simulink model "Lab2_Task_1"  (R2026a)
settings: Solver=FixedStepAuto  StopTime=inf
model workspace (MAT data in the model file):
  SL_ROS_VariableLengthArrays_MaxSizes.CommonInfo.ArrayTruncateAction = 'EmitWarning'
  SL_ROS_VariableLengthArrays_MaxSizes.MsgTypeMap = containers.Map
  SL_ROS_VariableLengthArrays_MaxSizes.MsgTypeMap.serialization.keys = {'sensor_msgs/LaserScan'}
  SL_ROS_VariableLengthArrays_MaxSizes.MsgTypeMap.serialization.values{1}(1).PropertyName = 'intensities'
  SL_ROS_VariableLengthArrays_MaxSizes.MsgTypeMap.serialization.values{1}(1).DataType = 'single'
  SL_ROS_VariableLengthArrays_MaxSizes.MsgTypeMap.serialization.values{1}(1).MaxLength = 360
  SL_ROS_VariableLengthArrays_MaxSizes.MsgTypeMap.serialization.values{1}(2).PropertyName = 'ranges'
  SL_ROS_VariableLengthArrays_MaxSizes.MsgTypeMap.serialization.values{1}(2).DataType = 'single'
  SL_ROS_VariableLengthArrays_MaxSizes.MsgTypeMap.serialization.values{1}(2).MaxLength = 360
  SL_ROS_VariableLengthArrays_MaxSizes.MsgTypeMap.serialization.uniformity = 0
  SL_ROS_VariableLengthArrays_MaxSizes.MsgTypeMap.serialization.keyType = 'char'
  SL_ROS_VariableLengthArrays_MaxSizes.MsgTypeMap.serialization.valueType = 'any'
undefined symbols (not defined in the file): header, twist
libraries: ros2lib x4
settings Model: Creator=scott  LastModifiedBy=juulg
settings OptimizationCC: PassReuseOutputArgsThreshold=0.0
settings HardwareCC: ProdHWDeviceType=Intel->x86-32 (Windows32)  UseEmbeddedCoderFeatures=off
settings RTWCC: SystemTargetFile=ert.tlc  HardwareBoard=Robot Operating System 2 (ROS 2)  TLCOptions="-aInlineSetEventsForThisBaseRateFcn=TLC_FALSE -aSuppressMultiTaskScheduler=TLC_FALSE  -aRateBasedStepFcn=0"  Toolchain=Colcon Tools  TargetLang=C++  Description=Embedded Coder
settings ERTTargetCC: ExtModeTransport=2.0  ExtModeAutomaticAllocSize=off  RootIOFormat=Structure reference  ERTCustomFileBanners=off  CodeInterfacePackaging=C++ class  SupportContinuousTime=on  SupportNonInlinedSFcns=on  ModelStepFunctionPrototypeControlCompliant=off

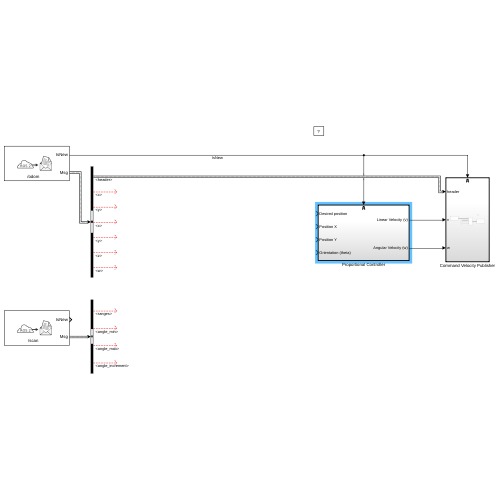
[thumbnail: Simulink's stored preview of the top-level diagram]
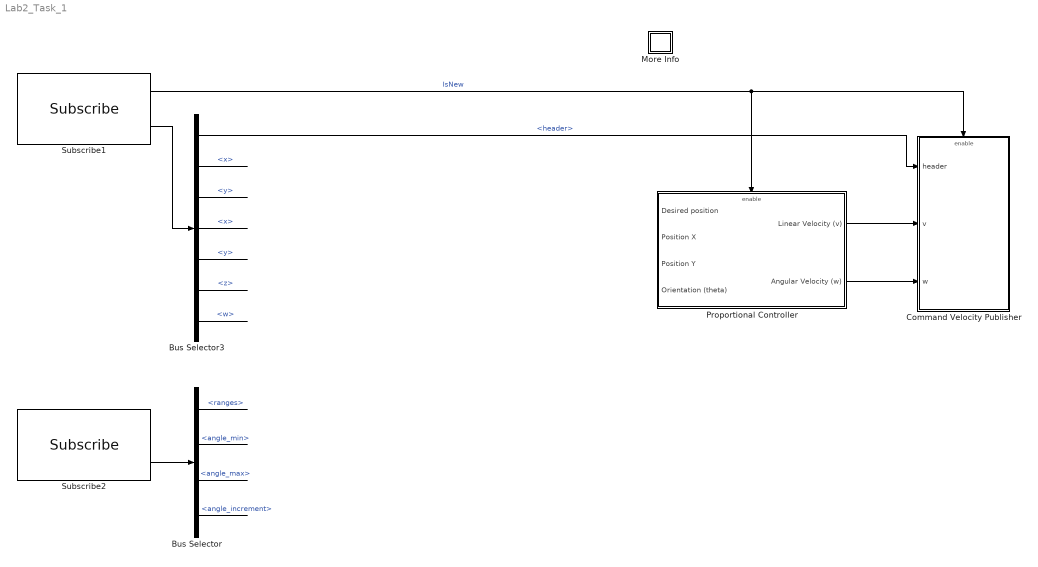
== system Lab2_Task_1 ==
  Bus Selector : BusSelector  OutputSignals=ranges,angle_min,angle_max,angle_increment
  Bus Selector3 : BusSelector  OutputSignals=header,pose.pose.position.x,pose.pose.position.y,pose.pose.orientation.x,pose.pose.orientation.y,pose.pose.orientation.z,pose.pose.orientation.w
  Command Velocity Publisher : Subsystem
  More Info : Subsystem
      settings: OpenFcn=showdemo(bdroot(gcb))
      mask Display: disp('?')
  Proportional Controller : Subsystem
  Subscribe1 : ros2lib/Subscribe  topicSource=Select from ROS network  topic=/odom  messageType=nav_msgs/Odometry  sampleTime=-1  QOSHistory=Keep last  QOSDepth=10  QOSReliability=Reliable  QOSDurability=Volatile  QOSDeadline=Inf  QOSLifespan=Inf  QOSLiveliness=Automatic  QOSLeaseDuration=Inf  QOSAvoidROSNamespaceConventions=off
  Subscribe2 : ros2lib/Subscribe  topicSource=Select from ROS network  topic=/scan  messageType=sensor_msgs/LaserScan  sampleTime=-1  QOSHistory=Keep last  QOSDepth=10  QOSReliability=Best effort  QOSDurability=Volatile  QOSDeadline=Inf  QOSLifespan=Inf  QOSLiveliness=Automatic  QOSLeaseDuration=Inf  QOSAvoidROSNamespaceConventions=off
  wires:
  Subscribe1/2 -> Bus Selector3/1
  Subscribe1/1 -> Command Velocity Publisher/Enable, Proportional Controller/Enable  "IsNew"
  Proportional Controller/1(Linear Velocity (v)) -> Command Velocity Publisher/2(v)
  Proportional Controller/2(Angular Velocity (w)) -> Command Velocity Publisher/3(w)
  Bus Selector3/1 -> Command Velocity Publisher/1(header)  "<header>"
  Bus Selector3/2 -> ?  "<x>"
  Bus Selector3/3 -> ?  "<y>"
  Bus Selector3/4 -> ?  "<x>"
  Bus Selector3/5 -> ?  "<y>"
  Bus Selector3/6 -> ?  "<z>"
  Bus Selector3/7 -> ?  "<w>"
  Subscribe2/2 -> Bus Selector/1
  Bus Selector/1 -> ?  "<ranges>"
  Bus Selector/2 -> ?  "<angle_min>"
  Bus Selector/3 -> ?  "<angle_max>"
  Bus Selector/4 -> ?  "<angle_increment>"

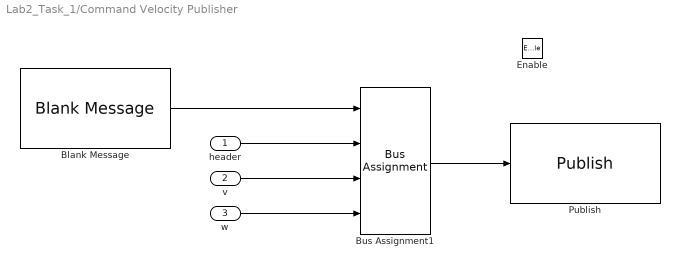
== system Lab2_Task_1/Command Velocity Publisher ==
  header : Inport
  v : Inport  Port=2
  w : Inport  Port=3
  Enable : EnablePort
  Blank Message : ros2lib/Blank Message  messageClass=Message  entityType=geometry_msgs/TwistStamped  messageType=geometry_msgs/TwistStamped  SampleTime=inf
  Bus Assignment1 : BusAssignment  DialogController=Simulink.DDGSource_BusAssignment  AssignedSignals=header,twist.linear.x,twist.angular.z
  Publish : ros2lib/Publish  topicSource=Select from ROS network  topic=/cmd_vel  messageType=geometry_msgs/TwistStamped  QOSHistory=Keep last  QOSDepth=10  QOSReliability=Reliable  QOSDurability=Volatile  QOSDeadline=Inf  QOSLifespan=Inf  QOSLiveliness=Automatic  QOSLeaseDuration=Inf  QOSAvoidROSNamespaceConventions=off
  wires:
  Bus Assignment1/1 -> Publish/1
  Blank Message/1 -> Bus Assignment1/1
  header/1 -> Bus Assignment1/2
  v/1 -> Bus Assignment1/3
  w/1 -> Bus Assignment1/4

== system Lab2_Task_1/More Info ==

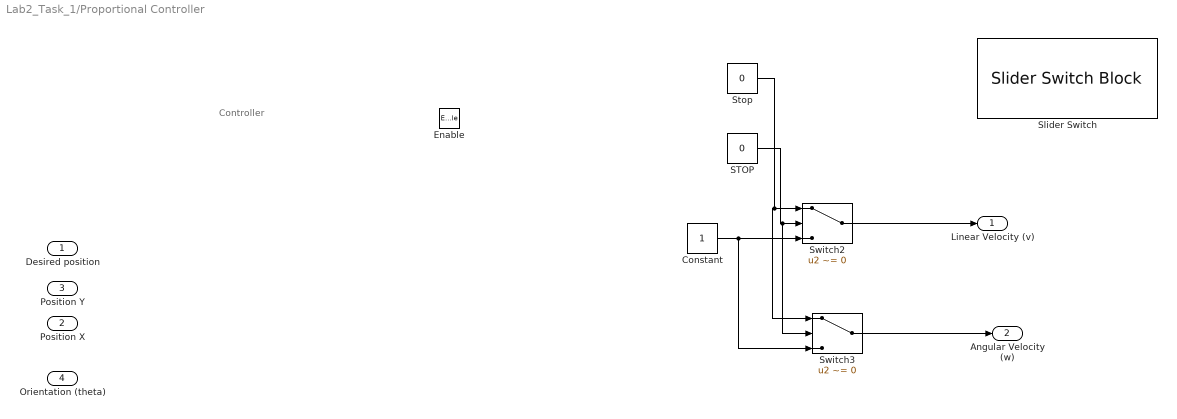
== system Lab2_Task_1/Proportional Controller ==
  note: Controller
  Desired position : Inport
  Position X : Inport  Port=2
  Position Y : Inport  Port=3
  Orientation (theta) : Inport  Port=4
  Enable : EnablePort
  Constant : Constant
  "STOP " : Constant  Value=0
  Slider Switch : SliderSwitchBlock
  Stop : Constant  Value=0
  Switch2 : Switch  Criteria=u2 ~= 0  SaturateOnIntegerOverflow=off  InputSameDT=off
  Switch3 : Switch  Criteria=u2 ~= 0  SaturateOnIntegerOverflow=off  InputSameDT=off
  Linear Velocity (v) : Outport  VectorParamsAs1DForOutWhenUnconnected=off
  Angular Velocity (w) : Outport  Port=2  VectorParamsAs1DForOutWhenUnconnected=off
  wires:
  Stop/1 -> Switch3/1, Switch2/1
  "STOP "/1 -> Switch3/2, Switch2/2
  Switch2/1 -> Linear Velocity (v)/1
  Switch3/1 -> Angular Velocity (w)/1
  Constant/1 -> Switch3/3, Switch2/3
